simulink model "Driver_test_sim"  (R2025b)
settings: Solver=FixedStepDiscrete  StartTime=0.0  StopTime=69.2  FixedStep=Ts  RelTol=1e-3
PreLoadFcn:
  | controller_params
InitFcn:
  | controller_params
values from neighbouring files (symbols this model uses):
  vBias = 0.3    [analyse_driver.m]
undefined symbols (not defined in the file or in its folder): Ao, Bo, DiscIntNeverNeededParam, K, Ke, plantD, tExc, Ts, vMax
libraries: simulink x1
settings Model: Creator=havard  LastModifiedBy=havard

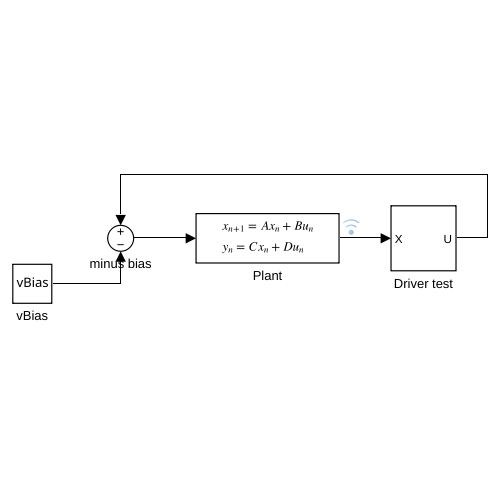
[thumbnail: Simulink's stored preview of the top-level diagram]
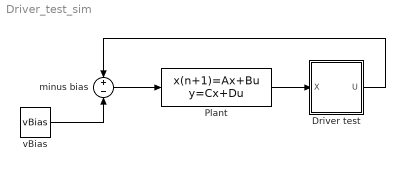
== system Driver_test_sim ==
  Driver test : Subsystem
  Plant : DiscreteStateSpace  A=plantD.A  B=plantD.B  C=plantD.C  D=0  SampleTime=Ts
  minus bias : Sum  Inputs=+-
  vBias : Constant  Value=vBias
  wires:
  Driver test/1(U) -> minus bias/1
  Plant/1 -> Driver test/1(X)
  minus bias/1 -> Plant/1
  vBias/1 -> minus bias/2

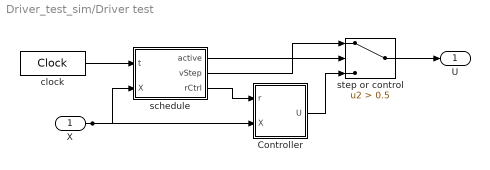
== system Driver_test_sim/Driver test ==
  X : Inport
  Controller : Subsystem
  clock : DigitalClock  SampleTime=Ts
  schedule : MATLAB Function  TreatAsAtomicUnit=on
  step or control : Switch  Criteria=u2 > Threshold  Threshold=0.5  SaturateOnIntegerOverflow=off  InputSameDT=off
  U : Outport
  wires:
  clock/1 -> schedule/1(t)
  X/1 -> Controller/2(X), schedule/2(X)
  step or control/1 -> U/1
  schedule/1(active) -> step or control/2
  schedule/2(vStep) -> step or control/1
  Controller/1(U) -> step or control/3
  schedule/3(rCtrl) -> Controller/1(r)

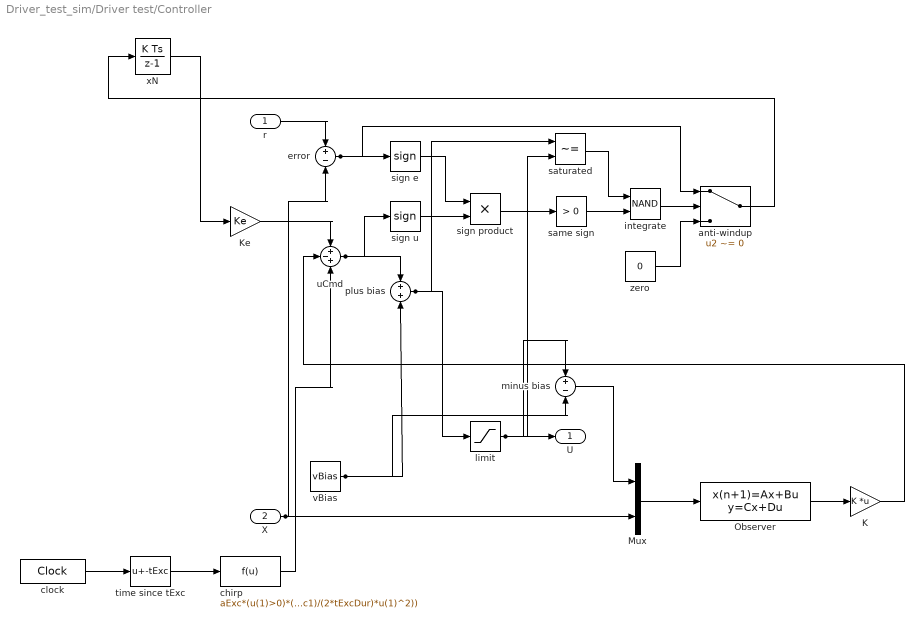
== system Driver_test_sim/Driver test/Controller ==
  r : Inport
  X : Inport  Port=2
  K : Gain  Gain=K  Multiplication=Matrix(K*u)
  Ke : Gain  Gain=Ke
  Mux : Mux  Inputs=2
  Observer : DiscreteStateSpace  A=Ao  B=Bo  C=eye(5)  D=zeros(5, 2)  SampleTime=Ts
  anti-windup : Switch  Criteria=u2 ~= 0  SaturateOnIntegerOverflow=off  InputSameDT=off
  chirp : Fcn  Expr=aExc*(u(1)>0)*(u(1)<tExcDur)*sin(2*pi*(fExc1*u(1) + (fExc2-fExc1)/(2*tExcDur)*u(1)^2))
  clock : DigitalClock  SampleTime=Ts
  error : Sum  Inputs=+-
  integrate : Logic  Operator=NAND  AllPortsSameDT=off  OutDataTypeStr=boolean
  limit : Saturate  UpperLimit=vMax  LowerLimit=-vMax
  minus bias : Sum  Inputs=+-
  plus bias : Sum
  same sign : simulink/Logic and Bit Operations/Compare To Constant  relop=>  const=0  OutDataTypeStr=boolean
  saturated : RelationalOperator  Operator=~=  OutDataTypeStr=boolean  RndMeth=Simplest  InputSameDT=off
  sign e : Signum
  sign product : Product
  sign u : Signum
  time since tExc : Bias  Bias=-tExc  SaturateOnIntegerOverflow=off
  uCmd : Sum  Inputs=+-+
  vBias : Constant  Value=vBias
  xN : DiscreteIntegrator  SampleTime=Ts  ICPrevOutput=DiscIntNeverNeededParam  ICPrevScaledInput=DiscIntNeverNeededParam
  zero : Constant  Value=0
  U : Outport
  wires:
  K/1 -> uCmd/2
  Observer/1 -> K/1
  integrate/1 -> anti-windup/2
  minus bias/1 -> Mux/1
  anti-windup/1 -> xN/1
  same sign/1 -> integrate/2
  limit/1 -> saturated/2, U/1, minus bias/1
  sign product/1 -> same sign/1
  clock/1 -> time since tExc/1
  Ke/1 -> uCmd/1
  X/1 -> error/2, Mux/2
  time since tExc/1 -> chirp/1
  chirp/1 -> uCmd/3
  zero/1 -> anti-windup/3
  error/1 -> sign e/1, anti-windup/1
  vBias/1 -> plus bias/2, minus bias/2
  saturated/1 -> integrate/1
  uCmd/1 -> sign u/1, plus bias/1
  r/1 -> error/1
  sign e/1 -> sign product/1
  Mux/1 -> Observer/1
  xN/1 -> Ke/1
  sign u/1 -> sign product/2
  plus bias/1 -> limit/1, saturated/1

== matlab function Driver_test_sim/Driver test/schedule ==
  data: t input; active output; X input; vStep output; rCtrl output
function [active, vStep, rCtrl] = schedule(t, X)
[active, vStep, rCtrl] = driver_schedule(t, X);
